simulink model "ps_isop_rail"  (R2026a)
settings: Solver=ode23tb  StopTime=param.sim.simlength  FixedStep=param.glb_time.tc  MaxStep=param.glb_time.tc
values from neighbouring files (symbols this model uses):
  param = struct()    [init_model.m]
libraries: fl_lib x49, nesl_utility x38, full_bridge_ideal_switch x4, single_phase_transformer x4, pi_ctrl x3, full_bridge_diode_rectifier x2, lithium_ion_battery x1, full_bridge_zvs_pwm_modulator x1, discrete_time_low_pass_filter x1
(part 1 of 2)
settings Model: SimulationMode=accelerator  Creator=dbagn  LastModifiedBy=dbagn
settings SolverCC: NumberNewtonIterations=3.0  ZeroCrossControl=DisableAll  SolverResetMethod=Robust
settings SFSimCC: CustomCodeUndefinedFunction=ThrowError  DefaultCustomCodeDeterministicFunctions=All
settings SFSimCC: SimCustomHeaderCode=|
  | #include "rpi.h"
  | #include "mavgflt.h"
  | #include "mavgflt_simulink.h"
  | #include "mavgflts.h"
  | #include "mavgflts_simulink.h"
  | #include "dsmavgflt.h"
  | #include "dsmavgflt_simulink.h"
  | #include "bemf_obsv.h"
  | #include "bemf_obsv_simulink.h"
  | #include "bemf_obsv_load_est.h"
  | #include "bemf_obsv_load_est_simulink.h"
  | #include "dqvector_pi.h"
  | #include "dqvector_pi_simulink.h"
  | #include "sv_pwm_simulink.h"
  | #include "sv_pwm.h"
  | #include "sv_pwm_cm_simulink.h"
  | #include "sv_pwm_cm.h"
  | #include "first_harmonic_tracker.h"
  | #include "first_harmonic_tracker_simulink.h"
  | #include "dqpll_thyr.h"
  | #include "dqpll_thyr_simulink.h"
  | #include "dqpll_grid.h"
  | #include "dqpll_grid_simulink.h"
  | #include "linear_double_integrator_observer_simulink.h"
  | #include "linear_double_integrator_observer.h"
settings SFSimCC: SimUserSources=|
  | "rpi.c"
  | "mavgflt_simulink.c"
  | "mavgflt.c"
  | "mavgflts_simulink.c"
  | "mavgflts.c"
  | "dsmavgflt_simulink.c"
  | "dsmavgflt.c"
  | "bemf_obsv_simulink.c"
  | "bemf_obsv.c"
  | "bemf_obsv_load_est_simulink.c"
  | "bemf_obsv_load_est.c"
  | "dqvector_pi.c"
  | "dqvector_pi_simulink.c"
  | "sv_pwm_simulink.c"
  | "sv_pwm.c"
  | "sv_pwm_cm_simulink.c"
  | "sv_pwm_cm.c"
  | "first_harmonic_tracker_simulink.c"
  | "first_harmonic_tracker.c"
  | "dqpll_thyr_simulink.c"
  | "dqpll_thyr.c"
  | "dqpll_grid_simulink.c"
  | "dqpll_grid.c"
  | "linear_double_integrator_observer_simulink.c"
  | "linear_double_integrator_observer.c"
settings SFSimCC: SimUserIncludeDirs=|
  | include
  | src
settings SimscapeCC: SimscapeNominalValues="[{\"value\":\"1\",\"unit\":\"A\"},{\"value\":\"1\",\"unit\":\"bar\"},{\"value\":\"1\",\"unit\":\"cm^2\"},{\"value\":\"1\",\"unit\":\"cm^3/s\"},{\"value\":\"1\",\"unit\":\"kJ/kg\"},{\"value\":\"1\",\"unit\":\"kW\"},{\"value\":\"1\",\"unit\":\"l\"},{\"value\":\"1\",\"unit\":\"N\"},{\"value\":\"1\",\"unit\":\"N*m\"},{\"value\":\"1\",\"unit\":\"V\"}]"  SimscapeLogType=none  SimscapeLogDataHistory=5000.0

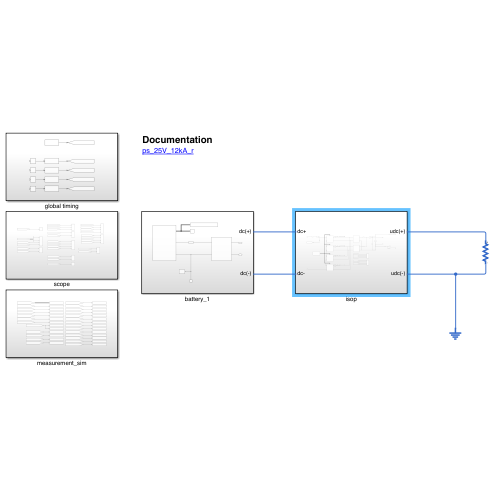
[thumbnail: Simulink's stored preview of the top-level diagram]
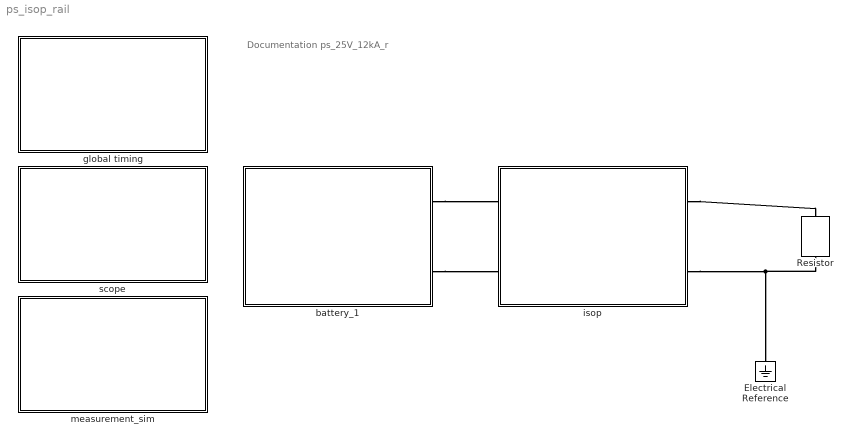
== system ps_isop_rail ==
  note: Documentation
      | ps_25V_12kA_r
  Electrical Reference : fl_lib/Electrical/Electrical Elements/Electrical Reference
  Resistor : fl_lib/Electrical/Electrical Elements/Resistor  R=param.load.rload Ohm  i_specify=off  i_priority=None  i=0 A  i_nominal_specify=off  i_nominal_value=1  i_nominal_unit=A  v_specify=off  v_priority=None  v=0 V  v_nominal_specify=off  v_nominal_value=1  v_nominal_unit=V
  battery_1 : Subsystem
  global timing : Subsystem
  isop : Subsystem
  measurement_sim : Subsystem
  scope : Subsystem
  connections:
  Resistor/RConn1 -- isop/RConn2 -- Electrical Reference/LConn1
  battery_1/RConn1 -- isop/LConn1
  battery_1/RConn2 -- isop/LConn2
  isop/RConn1 -- Resistor/LConn1

== system ps_isop_rail/battery_1 ==
  Electrical Reference : fl_lib/Electrical/Electrical Elements/Electrical Reference
  Inductor : fl_lib/Electrical/Electrical Elements/Inductor  l=param.battery.L_line H  r=0 Ohm  g=1e-9 1/Ohm  i_specify=off  i_priority=None  i=0 A  i_nominal_specify=off  i_nominal_value=1  i_nominal_unit=A  v_specify=off  v_priority=None  v=0 V  v_nominal_specify=off  v_nominal_value=1  v_nominal_unit=V  i_L_specify=off  i_L_priority=High  i_L=0 A  i_L_nominal_specify=off  i_L_nominal_value=1  i_L_nominal_unit=A
  Solver Configuration : nesl_utility/Solver Configuration  PhysicalDomain=network_engine_domain  SubClassName=solver  LeftPortType=input  RightPortType=generic  Tones=[]  Harmonics=[]  SimulateNoise=off  Profile=off  UseLocalSampling=off  EnableSwitchedLinearOptims=on  FrequencyDomain=off  UseCCode=off  RelTol=0.001  AbsTol=0.001  MinStep=1e-09  ToWorkspace=off  RevertToSquareIcSolve=off  NumHomotopyIterations=100  PhasorMode=off  PhasorModeNumHarmonics=1  ConsistencySolver=NEWTON_FTOL  CanonicalOrdering=UNORDERED  OptimizeIntermediates=UNOPTIMIZED  IndexReductionMethod=DerivativeReplacement  DoDC=on  ResidualTolerance=1e-3  ConsistencyTolSource=GLOBAL  ConsistencyAbsTol=0.001  ConsistencyRelTol=0.001  ConsistencyTolFactor=0.001  UseLocalSolver=on  LocalSolverChoice=NE_BACKWARD_EULER_ADVANCER  ResolveIndetEquations=on  FunctionEvalNumThread=1  LocalSolverSampleTime=param.glb_time.tc  DoFixedCost=on  MaxNonlinIter=param.sim.nonlinear_iterations  MaxModeIter=2  ComputeImpulses=off  ImpulseIterations=2  LinearAlgebra=auto  LinearAlgebraNumThread=0  EquationFormulation=NE_TIME_EF  DelaysMemoryBudget=1024  AutomaticFiltering=on  FilteringTimeConstant=0.001  PartitionStorageMethod=AS_NEEDED  PartitionMemoryBudget=1024  PartitionMethod=ROBUST  MultibodyUseLocalSolver=off  MultibodyLocalSolverChoice=ODE1  MultibodyLocalSolverSampleTime=0.001
  To Workspace14 : ToWorkspace  VariableName=battery_1_data_sim  SampleTime=param.glb_time.tc
      settings: MaxDataPoints=param.glb_time.Nc  Decimation=param.glb_time.decimation_tc
  lithium ion battery : Scope
      settings: ActiveDisplayYMinimum=-808.27997881012811  ActiveDisplayYMaximum=1287.7546757937268  DataLoggingVariableName=ScopeData3
  lithium_ion_battery : lithium_ion_battery/lithium_ion_battery  Q=param.battery.pack_1.Q  number_of_cells=param.battery.pack_1.number_of_cells  E_1=param.battery.pack_1.E_1  E0=param.battery.pack_1.E0  E1=param.battery.pack_1.E1  E2=param.battery.pack_1.E2  E3=param.battery.pack_1.E3  Elog=param.battery.pack_1.Elog  R0=param.battery.pack_1.R0  R1=param.battery.pack_1.R1  C1=param.battery.pack_1.C1  M=param.battery.pack_1.M  alpha=param.battery.pack_1.alpha  soc_init=param.battery.pack_1.soc_init  ts_battery=param.glb_time.ts_dab  q1Kalman=param.battery.pack_1.q1Kalman  q2Kalman=param.battery.pack_1.q2Kalman  q3Kalman=param.battery.pack_1.q3Kalman  rKalman=param.battery.pack_1.rKalman  tc=param.glb_time.tc  enable_white_noise_m=0
  single_phase_ui_measure : Subsystem
  dc(+) : PMIOPort  Side=Right
  dc(-) : PMIOPort  Port=2  Side=Right
  wires:
  lithium_ion_battery/1 -> To Workspace14/1, lithium ion battery/1
  connections:
  Solver Configuration/RConn1 -- lithium_ion_battery/RConn2 -- single_phase_ui_measure/LConn2 -- Electrical Reference/LConn1
  single_phase_ui_measure/RConn1 -- dc(+)/RConn1
  Inductor/LConn1 -- lithium_ion_battery/RConn1
  dc(-)/RConn1 -- single_phase_ui_measure/RConn2
  single_phase_ui_measure/LConn1 -- Inductor/RConn1

== system ps_isop_rail/global timing ==
  Unit Delay{1..4} (4 alike) : UnitDelay  SampleTime=param.glb_time.tc
  time_fbc1 : Subsystem  mask{k=1}
      mask prompts: k "Time Gain"
      mask Display:
      | disp('time-gen');
      | port_label('input', 1, 'crt');
      | port_label('output', 1, 'tout');
  time_fbc2 : Subsystem  mask{k=1}
      mask prompts: k "Time Gain"
      mask Display:
      | disp('time-gen');
      | port_label('input', 1, 'crt');
      | port_label('output', 1, 'tout');
  time_fbc3 : Subsystem  mask{k=1}
      mask prompts: k "Time Gain"
      mask Display:
      | disp('time-gen');
      | port_label('input', 1, 'crt');
      | port_label('output', 1, 'tout');
  time_fbc4 : Subsystem  mask{k=1}
      mask prompts: k "Time Gain"
      mask Display:
      | disp('time-gen');
      | port_label('input', 1, 'crt');
      | port_label('output', 1, 'tout');
  time_master : Subsystem  mask{k=1}
      mask prompts: k "Time Gain"
      mask Display:
      | disp('time-gen');
      | port_label('output', 1, 'tout');
  tag scope: time_isop_rail_module_1=global, time_isop_rail_module_2=global, time_isop_rail_module_3=global, time_isop_rail_module_4=global, time_master=global
  wires:
  time_master/1(Out1) -> [time_master]
  Unit Delay4/1 -> time_fbc1/1(correction_time)
  time_fbc1/1(Out1) -> [time_isop_rail_module_1]
  time_fbc2/1(Out1) -> [time_isop_rail_module_2]
  Unit Delay1/1 -> time_fbc2/1(correction_time)
  Unit Delay2/1 -> time_fbc3/1(correction_time)
  time_fbc3/1(Out1) -> [time_isop_rail_module_3]
  time_fbc4/1(Out1) -> [time_isop_rail_module_4]
  Unit Delay3/1 -> time_fbc4/1(correction_time)

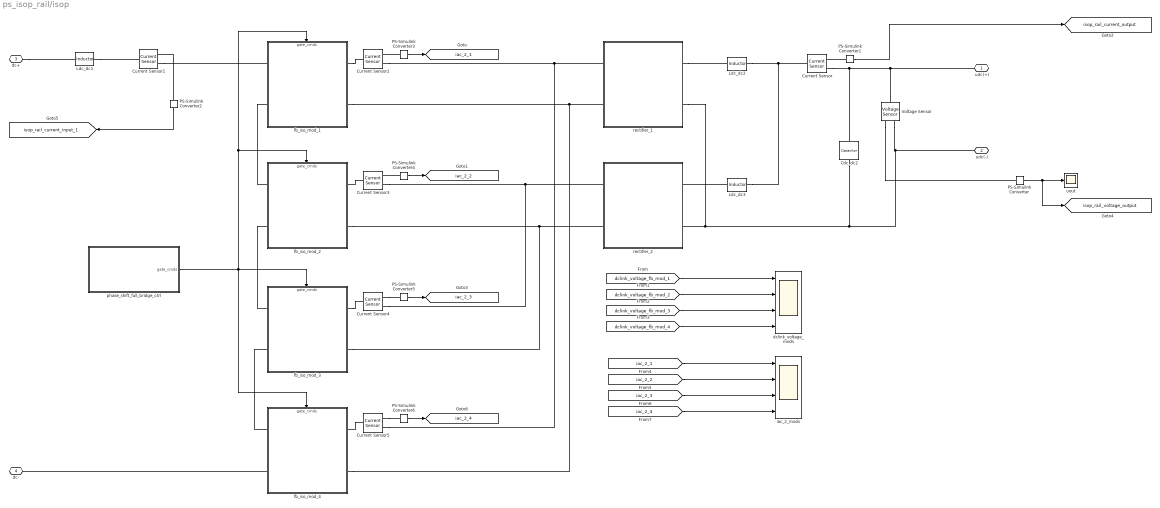
== system ps_isop_rail/isop ==
  Cdc_dc2 : fl_lib/Electrical/Electrical Elements/Capacitor  c=param.isop_rail.hw.Cdc_dc2 F  r=param.isop_rail.hw.RCdc_dc2 Ohm  g=0 1/Ohm  i_specify=off  i_priority=None  i=0 A  i_nominal_specify=off  i_nominal_value=1  i_nominal_unit=A  v_specify=off  v_priority=None  v=0 V  v_nominal_specify=off  v_nominal_value=1  v_nominal_unit=V  vc_specify=off  vc_priority=High  vc=0 V  vc_nominal_specify=off  vc_nominal_value=1  vc_nominal_unit=V
  Current Sensor{,1..5} (6 alike) : fl_lib/Electrical/Electrical Sensors/Current Sensor
  Ldc_dc1 : fl_lib/Electrical/Electrical Elements/Inductor  l=param.isop_rail.hw.Ldc_dc1 H  r=param.isop_rail.hw.RLdc_dc1 Ohm  g=1e-9 1/Ohm  i_specify=off  i_priority=None  i=0 A  i_nominal_specify=off  i_nominal_value=1  i_nominal_unit=A  v_specify=off  v_priority=None  v=0 V  v_nominal_specify=off  v_nominal_value=1  v_nominal_unit=V  i_L_specify=off  i_L_priority=High  i_L=0 A  i_L_nominal_specify=off  i_L_nominal_value=1  i_L_nominal_unit=A
  Ldc_dc2 : fl_lib/Electrical/Electrical Elements/Inductor  l=param.isop_rail.hw.Ldc_dc2 H  r=param.isop_rail.hw.RLdc_dc2 Ohm  g=1e-9 1/Ohm  i_specify=off  i_priority=None  i=0 A  i_nominal_specify=off  i_nominal_value=1  i_nominal_unit=A  v_specify=off  v_priority=None  v=0 V  v_nominal_specify=off  v_nominal_value=1  v_nominal_unit=V  i_L_specify=off  i_L_priority=High  i_L=0 A  i_L_nominal_specify=off  i_L_nominal_value=1  i_L_nominal_unit=A
  Ldc_dc3 : fl_lib/Electrical/Electrical Elements/Inductor  l=param.isop_rail.hw.Ldc_dc2 H  r=param.isop_rail.hw.RLdc_dc2 Ohm  g=1e-9 1/Ohm  i_specify=off  i_priority=None  i=0 A  i_nominal_specify=off  i_nominal_value=1  i_nominal_unit=A  v_specify=off  v_priority=None  v=0 V  v_nominal_specify=off  v_nominal_value=1  v_nominal_unit=V  i_L_specify=off  i_L_priority=High  i_L=0 A  i_L_nominal_specify=off  i_L_nominal_value=1  i_L_nominal_unit=A
  PS-Simulink Converter : nesl_utility/PS-Simulink Converter  PhysicalDomain=network_engine_domain  SubClassName=ps_output  LeftPortType=input  RightPortType=output  PseudoPeriodic=off  Frequencies=[]  VectorFormat=1-D array  Unit=V  AffineConversion=off
  PS-Simulink Converter{1..6} (6 alike) : nesl_utility/PS-Simulink Converter  PhysicalDomain=network_engine_domain  SubClassName=ps_output  LeftPortType=input  RightPortType=output  PseudoPeriodic=off  Frequencies=[]  VectorFormat=1-D array  Unit=A  AffineConversion=off
  Voltage Sensor : fl_lib/Electrical/Electrical Sensors/Voltage Sensor
  dclink_voltage_mods : Scope  NumInputPorts=4
      settings: ActiveDisplayYMinimum=1145.0339874920662  ActiveDisplayYMaximum=1193.3115786919072  DataLoggingVariableName=ScopeData4
  fb_iso_mod_1 : Subsystem
      settings: PortSchema="{\"entries\":[{\"content\":{\"sides\":[{\"content\":{\"connectorIds\":[\"In1\"]},\"type\":\"ConnectorPlacement.EquallySpacedRectSide\",\"uuid\":\"64125d2e-071e-4a4e-b242-e657f601aa6a\"},{\"content\":{\"side\":\"RIGHT\"},\"type\":\"ConnectorPlacement.EquallySpacedRectSide\",\"uuid\":\"9a259ce9-24e1-42ff-bc7d-5330e45b8a59\"},{\"content\":{\"connectorIds\":[\"LConn1\",\"LConn2\"],\"side\":\"TOP\"},\"type\":\"ConnectorPlacement.EquallySpacedRectSide\",\"uuid\":\"1c5aed3d-154a-406e-b3ed-8c68c35c38eb\"},{\"content\":{\"connectorIds\":[\"RConn1\",\"RConn2\"],\"side\":\"BOTTOM\"},\"type\":\"ConnectorPlacement.EquallySpacedRectSide\",\"uuid\":\"13746cdd-68e5-420a-ac86-8b06f3878da4\"}]},\"type\":\"ConnectorPlacement.EquallySpacedConnector\",\"uuid\":\"313792d0-2c30-49a3-9612-dddd30dbc396\"}],\"packageUris\":[\"http://schema.mathworks.com/mf0/Connector/R2020b\"],\"version\":\"1.0\"}"
  fb_iso_mod_2 : Subsystem
      settings: PortSchema="{\"entries\":[{\"content\":{\"sides\":[{\"content\":{\"connectorIds\":[\"In1\"]},\"type\":\"ConnectorPlacement.EquallySpacedRectSide\",\"uuid\":\"64125d2e-071e-4a4e-b242-e657f601aa6a\"},{\"content\":{\"side\":\"RIGHT\"},\"type\":\"ConnectorPlacement.EquallySpacedRectSide\",\"uuid\":\"9a259ce9-24e1-42ff-bc7d-5330e45b8a59\"},{\"content\":{\"connectorIds\":[\"LConn1\",\"LConn2\"],\"side\":\"TOP\"},\"type\":\"ConnectorPlacement.EquallySpacedRectSide\",\"uuid\":\"1c5aed3d-154a-406e-b3ed-8c68c35c38eb\"},{\"content\":{\"connectorIds\":[\"RConn1\",\"RConn2\"],\"side\":\"BOTTOM\"},\"type\":\"ConnectorPlacement.EquallySpacedRectSide\",\"uuid\":\"13746cdd-68e5-420a-ac86-8b06f3878da4\"}]},\"type\":\"ConnectorPlacement.EquallySpacedConnector\",\"uuid\":\"313792d0-2c30-49a3-9612-dddd30dbc396\"}],\"packageUris\":[\"http://schema.mathworks.com/mf0/Connector/R2020b\"],\"version\":\"1.0\"}"
  fb_iso_mod_3 : Subsystem
      settings: PortSchema="{\"entries\":[{\"content\":{\"sides\":[{\"content\":{\"connectorIds\":[\"In1\"]},\"type\":\"ConnectorPlacement.EquallySpacedRectSide\",\"uuid\":\"64125d2e-071e-4a4e-b242-e657f601aa6a\"},{\"content\":{\"side\":\"RIGHT\"},\"type\":\"ConnectorPlacement.EquallySpacedRectSide\",\"uuid\":\"9a259ce9-24e1-42ff-bc7d-5330e45b8a59\"},{\"content\":{\"connectorIds\":[\"LConn1\",\"LConn2\"],\"side\":\"TOP\"},\"type\":\"ConnectorPlacement.EquallySpacedRectSide\",\"uuid\":\"1c5aed3d-154a-406e-b3ed-8c68c35c38eb\"},{\"content\":{\"connectorIds\":[\"RConn1\",\"RConn2\"],\"side\":\"BOTTOM\"},\"type\":\"ConnectorPlacement.EquallySpacedRectSide\",\"uuid\":\"13746cdd-68e5-420a-ac86-8b06f3878da4\"}]},\"type\":\"ConnectorPlacement.EquallySpacedConnector\",\"uuid\":\"313792d0-2c30-49a3-9612-dddd30dbc396\"}],\"packageUris\":[\"http://schema.mathworks.com/mf0/Connector/R2020b\"],\"version\":\"1.0\"}"
  fb_iso_mod_4 : Subsystem
      settings: PortSchema="{\"entries\":[{\"content\":{\"sides\":[{\"content\":{\"connectorIds\":[\"In1\"]},\"type\":\"ConnectorPlacement.EquallySpacedRectSide\",\"uuid\":\"64125d2e-071e-4a4e-b242-e657f601aa6a\"},{\"content\":{\"side\":\"RIGHT\"},\"type\":\"ConnectorPlacement.EquallySpacedRectSide\",\"uuid\":\"9a259ce9-24e1-42ff-bc7d-5330e45b8a59\"},{\"content\":{\"connectorIds\":[\"LConn1\",\"LConn2\"],\"side\":\"TOP\"},\"type\":\"ConnectorPlacement.EquallySpacedRectSide\",\"uuid\":\"1c5aed3d-154a-406e-b3ed-8c68c35c38eb\"},{\"content\":{\"connectorIds\":[\"RConn1\",\"RConn2\"],\"side\":\"BOTTOM\"},\"type\":\"ConnectorPlacement.EquallySpacedRectSide\",\"uuid\":\"13746cdd-68e5-420a-ac86-8b06f3878da4\"}]},\"type\":\"ConnectorPlacement.EquallySpacedConnector\",\"uuid\":\"313792d0-2c30-49a3-9612-dddd30dbc396\"}],\"packageUris\":[\"http://schema.mathworks.com/mf0/Connector/R2020b\"],\"version\":\"1.0\"}"
  iac_2_mods : Scope  NumInputPorts=4
      settings: ActiveDisplayYMinimum=-468.571106856033  ActiveDisplayYMaximum=468.19314645491767  DataLoggingVariableName=ScopeData5
  phase_shift_full_bridge_ctrl : Subsystem
  rectifier_1 : Subsystem
  rectifier_2 : Subsystem
  uout : Scope
      settings: ActiveDisplayYMinimum=-94.552187389541785  ActiveDisplayYMaximum=850.96968650587621
  udc(+) : PMIOPort  Side=Right
  udc(-) : PMIOPort  Port=2  Side=Right
  dc+ : PMIOPort  Port=3  Side=Left
  dc- : PMIOPort  Port=4  Side=Left
  tag scope: iac_2_1=global, iac_2_2=global, iac_2_3=global, iac_2_4=global, isop_rail_current_input_1=global, isop_rail_current_output=global, isop_rail_voltage_output=global
  wires:
  phase_shift_full_bridge_ctrl/1(gate_cmds) -> fb_iso_mod_4/1(gate_cmds), fb_iso_mod_3/1(gate_cmds), fb_iso_mod_2/1(gate_cmds), fb_iso_mod_1/1(gate_cmds)
  PS-Simulink Converter/1 -> [isop_rail_voltage_output], uout/1
  [dclink_voltage_fb_mod_4] -> dclink_voltage_mods/4
  [dclink_voltage_fb_mod_3] -> dclink_voltage_mods/3
  [dclink_voltage_fb_mod_2] -> dclink_voltage_mods/2
  [dclink_voltage_fb_mod_1] -> dclink_voltage_mods/1
  PS-Simulink Converter1/1 -> [isop_rail_current_output]
  PS-Simulink Converter2/1 -> [isop_rail_current_input_1]
  PS-Simulink Converter3/1 -> [iac_2_1]
  PS-Simulink Converter4/1 -> [iac_2_2]
  PS-Simulink Converter5/1 -> [iac_2_3]
  PS-Simulink Converter6/1 -> [iac_2_4]
  [iac_2_4] -> iac_2_mods/4
  [iac_2_3] -> iac_2_mods/3
  [iac_2_2] -> iac_2_mods/2
  [iac_2_1] -> iac_2_mods/1
  connections:
  fb_iso_mod_2/LConn1 -- fb_iso_mod_1/LConn2
  fb_iso_mod_3/LConn1 -- fb_iso_mod_2/LConn2
  fb_iso_mod_4/LConn1 -- fb_iso_mod_3/LConn2
  fb_iso_mod_4/LConn2 -- dc-/RConn1
  Current Sensor3/RConn2 -- Current Sensor4/RConn2 -- rectifier_2/LConn1
  rectifier_2/LConn2 -- fb_iso_mod_3/RConn2 -- fb_iso_mod_2/RConn2
  Current Sensor2/RConn2 -- Current Sensor5/RConn2 -- rectifier_1/LConn1
  fb_iso_mod_1/RConn2 -- fb_iso_mod_4/RConn2 -- rectifier_1/LConn2
  udc(+)/RConn1 -- Current Sensor/RConn2 -- Cdc_dc2/LConn1 -- Voltage Sensor/LConn1
  dc+/RConn1 -- Ldc_dc1/LConn1
  Voltage Sensor/RConn1 -- PS-Simulink Converter/LConn1
  Ldc_dc2/RConn1 -- Ldc_dc3/RConn1 -- Current Sensor/LConn1
  PS-Simulink Converter1/LConn1 -- Current Sensor/RConn1
  Current Sensor1/RConn2 -- fb_iso_mod_1/LConn1
  Ldc_dc1/RConn1 -- Current Sensor1/LConn1
  PS-Simulink Converter2/LConn1 -- Current Sensor1/RConn1
  rectifier_1/RConn1 -- Ldc_dc2/LConn1
  Voltage Sensor/RConn2 -- rectifier_1/RConn2 -- rectifier_2/RConn2 -- Cdc_dc2/RConn1 -- udc(-)/RConn1
  Ldc_dc3/LConn1 -- rectifier_2/RConn1
  fb_iso_mod_1/RConn1 -- Current Sensor2/LConn1
  Current Sensor3/LConn1 -- fb_iso_mod_2/RConn1
  fb_iso_mod_3/RConn1 -- Current Sensor4/LConn1
  Current Sensor5/LConn1 -- fb_iso_mod_4/RConn1
  PS-Simulink Converter3/LConn1 -- Current Sensor2/RConn1
  PS-Simulink Converter4/LConn1 -- Current Sensor3/RConn1
  Current Sensor4/RConn1 -- PS-Simulink Converter5/LConn1
  Current Sensor5/RConn1 -- PS-Simulink Converter6/LConn1

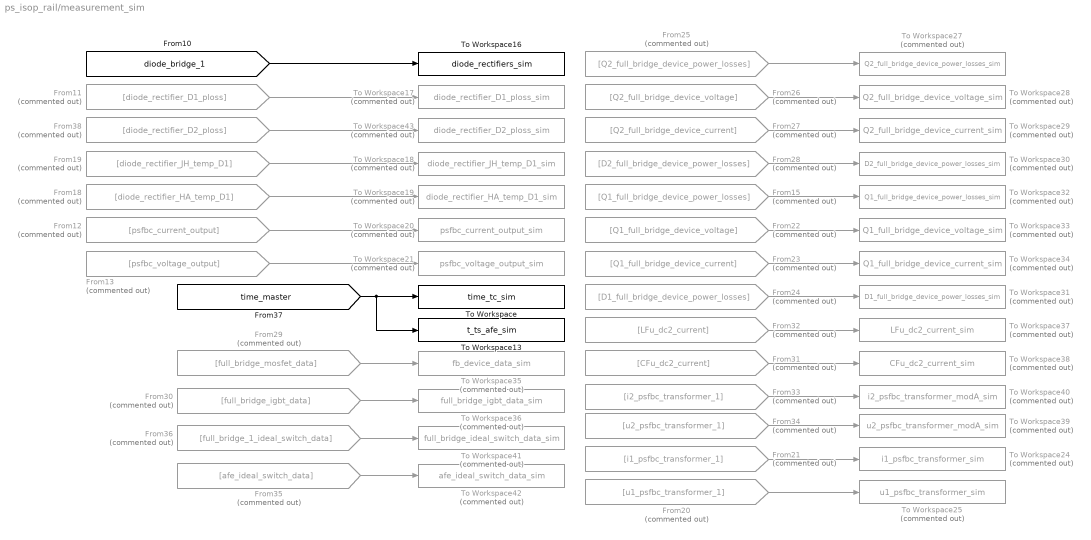
== system ps_isop_rail/measurement_sim ==
  From11 : From  Commented=on  GotoTag=diode_rectifier_D1_ploss
  From12 : From  Commented=on  GotoTag=psfbc_current_output
  From13 : From  Commented=on  GotoTag=psfbc_voltage_output
  From15 : From  Commented=on  GotoTag=Q1_full_bridge_device_power_losses
  From18 : From  Commented=on  GotoTag=diode_rectifier_HA_temp_D1
  From19 : From  Commented=on  GotoTag=diode_rectifier_JH_temp_D1
  From20 : From  Commented=on  GotoTag=u1_psfbc_transformer_1
  From21 : From  Commented=on  GotoTag=i1_psfbc_transformer_1
  From22 : From  Commented=on  GotoTag=Q1_full_bridge_device_voltage
  From23 : From  Commented=on  GotoTag=Q1_full_bridge_device_current
  From24 : From  Commented=on  GotoTag=D1_full_bridge_device_power_losses
  From25 : From  Commented=on  GotoTag=Q2_full_bridge_device_power_losses
  From26 : From  Commented=on  GotoTag=Q2_full_bridge_device_voltage
  From27 : From  Commented=on  GotoTag=Q2_full_bridge_device_current
  From28 : From  Commented=on  GotoTag=D2_full_bridge_device_power_losses
  From29 : From  Commented=on  GotoTag=full_bridge_mosfet_data
  From30 : From  Commented=on  GotoTag=full_bridge_igbt_data
  From31 : From  Commented=on  GotoTag=CFu_dc2_current
  From32 : From  Commented=on  GotoTag=LFu_dc2_current
  From33 : From  Commented=on  GotoTag=i2_psfbc_transformer_1
  From34 : From  Commented=on  GotoTag=u2_psfbc_transformer_1
  From35 : From  Commented=on  GotoTag=afe_ideal_switch_data
  From36 : From  Commented=on  GotoTag=full_bridge_1_ideal_switch_data
  From38 : From  Commented=on  GotoTag=diode_rectifier_D2_ploss
  To Workspace : ToWorkspace  VariableName=time_tc_sim  SampleTime=param.glb_time.tc
      settings: MaxDataPoints=param.glb_time.Nc  Decimation=param.glb_time.decimation_tc
  To Workspace13 : ToWorkspace  VariableName=t_ts_afe_sim  SampleTime=param.glb_time.ts_isop_rail
      settings: MaxDataPoints=param.glb_time.Ns_isop_rail
  To Workspace16 : ToWorkspace  VariableName=diode_rectifiers_sim  SampleTime=param.glb_time.tc
      settings: MaxDataPoints=param.glb_time.Nc  Decimation=param.glb_time.decimation_tc
  To Workspace17 : ToWorkspace  Commented=on  VariableName=diode_rectifier_D1_ploss_sim  SampleTime=param.glb_time.tc
      settings: MaxDataPoints=param.glb_time.Nc  Decimation=param.glb_time.decimation_tc
  To Workspace18 : ToWorkspace  Commented=on  VariableName=diode_rectifier_JH_temp_D1_sim  SampleTime=param.glb_time.tc
      settings: MaxDataPoints=param.glb_time.Nc  Decimation=param.glb_time.decimation_tc
  To Workspace19 : ToWorkspace  Commented=on  VariableName=diode_rectifier_HA_temp_D1_sim  SampleTime=param.glb_time.tc
      settings: MaxDataPoints=param.glb_time.Nc  Decimation=param.glb_time.decimation_tc
  To Workspace20 : ToWorkspace  Commented=on  VariableName=psfbc_current_output_sim  SampleTime=param.glb_time.tc
      settings: MaxDataPoints=param.glb_time.Nc  Decimation=param.glb_time.decimation_tc
  To Workspace21 : ToWorkspace  Commented=on  VariableName=psfbc_voltage_output_sim  SampleTime=param.glb_time.tc
      settings: MaxDataPoints=param.glb_time.Nc  Decimation=param.glb_time.decimation_tc
  To Workspace24 : ToWorkspace  Commented=on  VariableName=i1_psfbc_transformer_sim  SampleTime=param.glb_time.tc
      settings: MaxDataPoints=param.glb_time.Nc  Decimation=param.glb_time.decimation_tc
  To Workspace25 : ToWorkspace  Commented=on  VariableName=u1_psfbc_transformer_sim  SampleTime=param.glb_time.tc
      settings: MaxDataPoints=param.glb_time.Nc  Decimation=param.glb_time.decimation_tc
  To Workspace27 : ToWorkspace  Commented=on  VariableName=Q2_full_bridge_device_power_losses_sim  SampleTime=param.glb_time.tc
      settings: MaxDataPoints=param.glb_time.Nc  Decimation=param.glb_time.decimation_tc
  To Workspace28 : ToWorkspace  Commented=on  VariableName=Q2_full_bridge_device_voltage_sim  SampleTime=param.glb_time.tc
      settings: MaxDataPoints=param.glb_time.Nc  Decimation=param.glb_time.decimation_tc
  To Workspace29 : ToWorkspace  Commented=on  VariableName=Q2_full_bridge_device_current_sim  SampleTime=param.glb_time.tc
      settings: MaxDataPoints=param.glb_time.Nc  Decimation=param.glb_time.decimation_tc
  To Workspace30 : ToWorkspace  Commented=on  VariableName=D2_full_bridge_device_power_losses_sim  SampleTime=param.glb_time.tc
      settings: MaxDataPoints=param.glb_time.Nc  Decimation=param.glb_time.decimation_tc
  To Workspace31 : ToWorkspace  Commented=on  VariableName=D1_full_bridge_device_power_losses_sim  SampleTime=param.glb_time.tc
      settings: MaxDataPoints=param.glb_time.Nc  Decimation=param.glb_time.decimation_tc
  To Workspace32 : ToWorkspace  Commented=on  VariableName=Q1_full_bridge_device_power_losses_sim  SampleTime=param.glb_time.tc
      settings: MaxDataPoints=param.glb_time.Nc  Decimation=param.glb_time.decimation_tc
  To Workspace33 : ToWorkspace  Commented=on  VariableName=Q1_full_bridge_device_voltage_sim  SampleTime=param.glb_time.tc
      settings: MaxDataPoints=param.glb_time.Nc  Decimation=param.glb_time.decimation_tc
  To Workspace34 : ToWorkspace  Commented=on  VariableName=Q1_full_bridge_device_current_sim  SampleTime=param.glb_time.tc
      settings: MaxDataPoints=param.glb_time.Nc  Decimation=param.glb_time.decimation_tc
  To Workspace35 : ToWorkspace  Commented=on  VariableName=fb_device_data_sim  SampleTime=param.glb_time.tc
      settings: MaxDataPoints=param.glb_time.Nc  Decimation=param.glb_time.decimation_tc
  To Workspace36 : ToWorkspace  Commented=on  VariableName=full_bridge_igbt_data_sim  SampleTime=param.glb_time.tc
      settings: MaxDataPoints=param.glb_time.Nc  Decimation=param.glb_time.decimation_tc
  To Workspace37 : ToWorkspace  Commented=on  VariableName=LFu_dc2_current_sim  SampleTime=param.glb_time.tc
      settings: MaxDataPoints=param.glb_time.Nc  Decimation=param.glb_time.decimation_tc
  To Workspace38 : ToWorkspace  Commented=on  VariableName=CFu_dc2_current_sim  SampleTime=param.glb_time.tc
      settings: MaxDataPoints=param.glb_time.Nc  Decimation=param.glb_time.decimation_tc
  To Workspace39 : ToWorkspace  Commented=on  VariableName=u2_psfbc_transformer_modA_sim  SampleTime=param.glb_time.tc
      settings: MaxDataPoints=param.glb_time.Nc  Decimation=param.glb_time.decimation_tc
  To Workspace40 : ToWorkspace  Commented=on  VariableName=i2_psfbc_transformer_modA_sim  SampleTime=param.glb_time.tc
      settings: MaxDataPoints=param.glb_time.Nc  Decimation=param.glb_time.decimation_tc
  To Workspace41 : ToWorkspace  Commented=on  VariableName=full_bridge_ideal_switch_data_sim  SampleTime=param.glb_time.tc
      settings: MaxDataPoints=param.glb_time.Nc  Decimation=param.glb_time.decimation_tc
  To Workspace42 : ToWorkspace  Commented=on  VariableName=afe_ideal_switch_data_sim  SampleTime=param.glb_time.tc
      settings: MaxDataPoints=param.glb_time.Nc  Decimation=param.glb_time.decimation_tc
  To Workspace43 : ToWorkspace  Commented=on  VariableName=diode_rectifier_D2_ploss_sim  SampleTime=param.glb_time.tc
      settings: MaxDataPoints=param.glb_time.Nc  Decimation=param.glb_time.decimation_tc
  wires:
  [time_master] -> To Workspace13/1, To Workspace/1
  [diode_bridge_1] -> To Workspace16/1
  From19/1 -> To Workspace18/1
  From11/1 -> To Workspace17/1
  From18/1 -> To Workspace19/1
  From12/1 -> To Workspace20/1
  From13/1 -> To Workspace21/1
  From21/1 -> To Workspace24/1
  From20/1 -> To Workspace25/1
  From25/1 -> To Workspace27/1
  From26/1 -> To Workspace28/1
  From27/1 -> To Workspace29/1
  From15/1 -> To Workspace32/1
  From22/1 -> To Workspace33/1
  From23/1 -> To Workspace34/1
  From28/1 -> To Workspace30/1
  From24/1 -> To Workspace31/1
  From29/1 -> To Workspace35/1
  From30/1 -> To Workspace36/1
  From32/1 -> To Workspace37/1
  From31/1 -> To Workspace38/1
  From34/1 -> To Workspace39/1
  From33/1 -> To Workspace40/1
  From36/1 -> To Workspace41/1
  From35/1 -> To Workspace42/1
  From38/1 -> To Workspace43/1

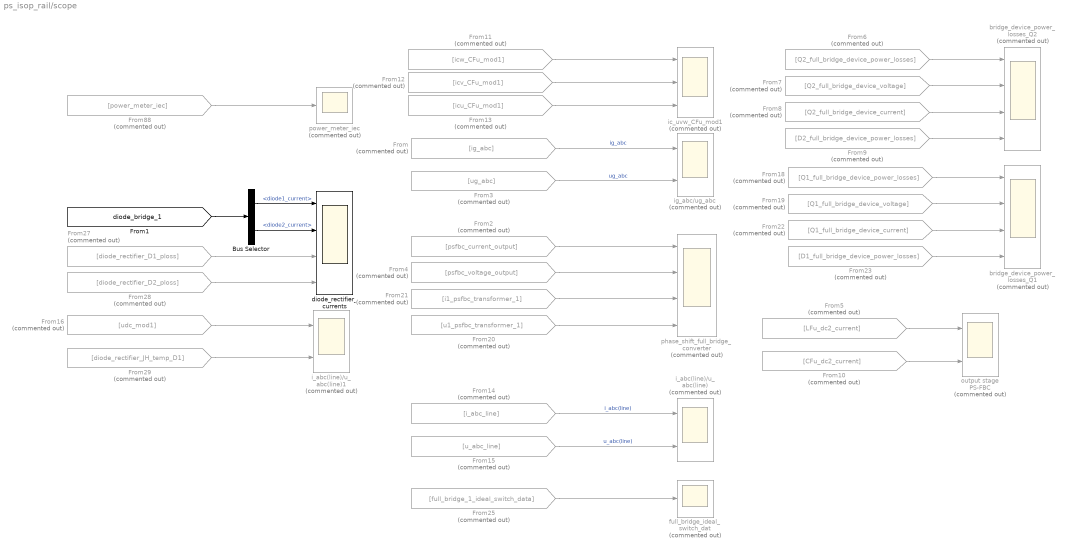
== system ps_isop_rail/scope ==
  Bus Selector : BusSelector  OutputSignals=diode1_current,diode2_current
  From : From  Commented=on  GotoTag=ig_abc
  From10 : From  Commented=on  GotoTag=CFu_dc2_current
  From11 : From  Commented=on  GotoTag=icw_CFu_mod1
  From12 : From  Commented=on  GotoTag=icv_CFu_mod1
  From13 : From  Commented=on  GotoTag=icu_CFu_mod1
  From14 : From  Commented=on  GotoTag=i_abc_line
  From15 : From  Commented=on  GotoTag=u_abc_line
  From16 : From  Commented=on  GotoTag=udc_mod1
  From18 : From  Commented=on  GotoTag=Q1_full_bridge_device_power_losses
  From19 : From  Commented=on  GotoTag=Q1_full_bridge_device_voltage
  From2 : From  Commented=on  GotoTag=psfbc_current_output
  From20 : From  Commented=on  GotoTag=u1_psfbc_transformer_1
  From21 : From  Commented=on  GotoTag=i1_psfbc_transformer_1
  From22 : From  Commented=on  GotoTag=Q1_full_bridge_device_current
  From23 : From  Commented=on  GotoTag=D1_full_bridge_device_power_losses
  From25 : From  Commented=on  GotoTag=full_bridge_1_ideal_switch_data
  From27 : From  Commented=on  GotoTag=diode_rectifier_D1_ploss
  From28 : From  Commented=on  GotoTag=diode_rectifier_D2_ploss
  From29 : From  Commented=on  GotoTag=diode_rectifier_JH_temp_D1
  From3 : From  Commented=on  GotoTag=ug_abc
  From4 : From  Commented=on  GotoTag=psfbc_voltage_output
  From5 : From  Commented=on  GotoTag=LFu_dc2_current
  From6 : From  Commented=on  GotoTag=Q2_full_bridge_device_power_losses
  From7 : From  Commented=on  GotoTag=Q2_full_bridge_device_voltage
  From8 : From  Commented=on  GotoTag=Q2_full_bridge_device_current
  From88 : From  Commented=on  GotoTag=power_meter_iec
  From9 : From  Commented=on  GotoTag=D2_full_bridge_device_power_losses
  bridge_device_power_losses_Q1 : Scope  Commented=on  NumInputPorts=4
      settings: SampleTime=param.glb_time.tc  ActiveDisplayYMinimum=-132.81353179927618  ActiveDisplayYMaximum=1178.2847224343986  DataLoggingVariableName=ScopeData23
  bridge_device_power_losses_Q2 : Scope  Commented=on  NumInputPorts=4
      settings: SampleTime=param.glb_time.tc  ActiveDisplayYMinimum=-102.91748468374873  ActiveDisplayYMaximum=909.22247743852836  DataLoggingVariableName=ScopeData20
  diode_rectifier_currents : Scope  NumInputPorts=4
      settings: ActiveDisplayString=3  ActiveDisplayYMinimum=15269.321807853252  ActiveDisplayYMaximum=15276.006477439711  DataLoggingVariableName=ScopeData11
  full_bridge_ideal_switch_dat : Scope  Commented=on
      settings: SampleTime=param.glb_time.tc  ActiveDisplayYMinimum=-185.80082711442992  ActiveDisplayYMaximum=1530.3864871069391  DataLoggingVariableName=ScopeData25
  i_abc(line)/u_abc(line) : Scope  Commented=on  NumInputPorts=2
      settings: SampleTime=param.glb_time.tc  ActiveDisplayYMinimum=-489.89794788487484  ActiveDisplayYMaximum=489.89794788490036  DataLoggingVariableName=ScopeData18
  i_abc(line)/u_abc(line)1 : Scope  Commented=on  NumInputPorts=2
      settings: SampleTime=param.glb_time.tc  ActiveDisplayYMinimum=-1  ActiveDisplayYMaximum=1  DataLoggingVariableName=ScopeData19
  ic_uvw_CFu_mod1 : Scope  Commented=on  NumInputPorts=3
      settings: SampleTime=param.glb_time.tc  ActiveDisplayYMinimum=-250.78571798939993  ActiveDisplayYMaximum=408.17461480787006  DataLoggingVariableName=ScopeData17
  ig_abc/ug_abc : Scope  Commented=on  NumInputPorts=2
      settings: SampleTime=param.glb_time.tc  ActiveDisplayYMinimum=-494.737319512461  ActiveDisplayYMaximum=494.80225542196177  DataLoggingVariableName=ScopeData15
  output stage PS-FBC : Scope  Commented=on  NumInputPorts=2
      settings: SampleTime=param.glb_time.tc  ActiveDisplayYMinimum=-658.65362756432182  ActiveDisplayYMaximum=664.76716339933853  DataLoggingVariableName=ScopeData22
  phase_shift_full_bridge_converter : Scope  Commented=on  NumInputPorts=4
      settings: SampleTime=param.glb_time.tc  ActiveDisplayYMinimum=-1597.686541193829  ActiveDisplayYMaximum=14379.178870744465  DataLoggingVariableName=ScopeData16
  power_meter_iec : Scope  Commented=on
      settings: SampleTime=param.glb_time.tc  ActiveDisplayYMinimum=-185.80082711442992  ActiveDisplayYMaximum=1530.3864871069391  DataLoggingVariableName=ScopeData27
  wires:
  From3/1 -> ig_abc/ug_abc/2  "ug_abc"
  From/1 -> ig_abc/ug_abc/1  "ig_abc"
  From11/1 -> ic_uvw_CFu_mod1/1
  From12/1 -> ic_uvw_CFu_mod1/2
  From13/1 -> ic_uvw_CFu_mod1/3
  From14/1 -> i_abc(line)/u_abc(line)/1  "i_abc(line)"
  From15/1 -> i_abc(line)/u_abc(line)/2  "u_abc(line)"
  From16/1 -> i_abc(line)/u_abc(line)1/1
  [diode_bridge_1] -> Bus Selector/1
  From2/1 -> phase_shift_full_bridge_converter/1
  From4/1 -> phase_shift_full_bridge_converter/2
  From21/1 -> phase_shift_full_bridge_converter/3
  From20/1 -> phase_shift_full_bridge_converter/4
  Bus Selector/1 -> diode_rectifier_currents/1  "<diode1_current>"
  Bus Selector/2 -> diode_rectifier_currents/2  "<diode2_current>"
  From5/1 -> output stage PS-FBC/1
  From10/1 -> output stage PS-FBC/2
  From6/1 -> bridge_device_power_losses_Q2/1
  From7/1 -> bridge_device_power_losses_Q2/2
  From8/1 -> bridge_device_power_losses_Q2/3
  From9/1 -> bridge_device_power_losses_Q2/4
  From18/1 -> bridge_device_power_losses_Q1/1
  From19/1 -> bridge_device_power_losses_Q1/2
  From22/1 -> bridge_device_power_losses_Q1/3
  From23/1 -> bridge_device_power_losses_Q1/4
  From25/1 -> full_bridge_ideal_switch_dat/1
  From27/1 -> diode_rectifier_currents/3
  From28/1 -> diode_rectifier_currents/4
  From29/1 -> i_abc(line)/u_abc(line)1/2
  From88/1 -> power_meter_iec/1

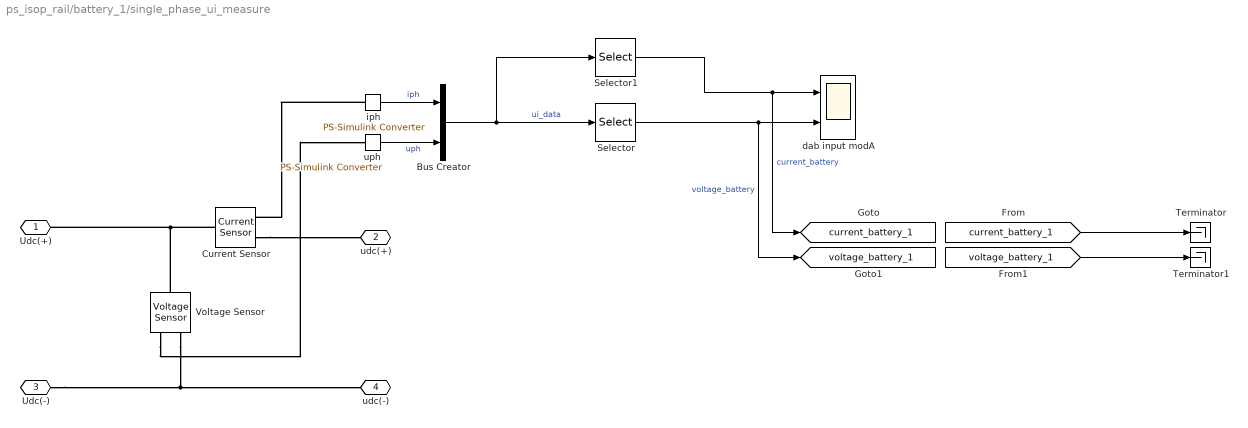
== system ps_isop_rail/battery_1/single_phase_ui_measure ==
  Bus Creator : BusCreator  Inputs=2
  Current Sensor : fl_lib/Electrical/Electrical Sensors/Current Sensor
  Selector : Selector  InputPortWidth=2  IndexOptions=Index vector (dialog)  Indices=2  OutputSizes=1
  Selector1 : Selector  InputPortWidth=2  IndexOptions=Index vector (dialog)  Indices=1  OutputSizes=1
  Terminator : Terminator
  Terminator1 : Terminator
  Voltage Sensor : fl_lib/Electrical/Electrical Sensors/Voltage Sensor
  dab input modA : Scope  NumInputPorts=2
      settings: SampleTime=param.glb_time.tc  ActiveDisplayYMinimum=4618.3089115716557  ActiveDisplayYMaximum=4703.2257607249676  DataLoggingVariableName=ScopeData2
  iph : nesl_utility/PS-Simulink Converter  PhysicalDomain=network_engine_domain  SubClassName=ps_output  LeftPortType=input  RightPortType=output  PseudoPeriodic=off  Frequencies=[]  VectorFormat=1-D array  Unit=A  AffineConversion=off
  uph : nesl_utility/PS-Simulink Converter  PhysicalDomain=network_engine_domain  SubClassName=ps_output  LeftPortType=input  RightPortType=output  PseudoPeriodic=off  Frequencies=[]  VectorFormat=1-D array  Unit=V  AffineConversion=off
  Udc(+) : PMIOPort  Side=Left
  udc(+) : PMIOPort  Port=2  Side=Right
  Udc(-) : PMIOPort  Port=3  Side=Left
  udc(-) : PMIOPort  Port=4  Side=Right
  tag scope: current_battery_1=global, voltage_battery_1=global
  wires:
  Bus Creator/1 -> Selector/1, Selector1/1  "ui_data"
  iph/1 -> Bus Creator/1  "iph"
  uph/1 -> Bus Creator/2  "uph"
  Selector1/1 -> [current_battery_1], dab input modA/1  "current_battery"
  Selector/1 -> dab input modA/2, [voltage_battery_1]  "voltage_battery"
  [current_battery_1] -> Terminator/1
  [voltage_battery_1] -> Terminator1/1
  connections:
  iph/LConn1 -- Current Sensor/RConn1
  Voltage Sensor/LConn1 -- Current Sensor/LConn1 -- Udc(+)/RConn1
  Current Sensor/RConn2 -- udc(+)/RConn1
  Voltage Sensor/RConn1 -- uph/LConn1
  Voltage Sensor/RConn2 -- Udc(-)/RConn1 -- udc(-)/RConn1

== system ps_isop_rail/global timing/time_fbc1 ==
  correction_time : Inport
  Constant : Constant
  Gain : Gain  Gain=k
  Product : Product
  Sum : Sum  Inputs=|++
  time_1 : Clock
  Out1 : Outport
  wires:
  Sum/1 -> Product/2
  Constant/1 -> Sum/2
  correction_time/1 -> Sum/1
  Product/1 -> Out1/1
  Gain/1 -> Product/1
  time_1/1 -> Gain/1

== system ps_isop_rail/global timing/time_fbc2 ==
  correction_time : Inport
  Constant : Constant
  Gain : Gain  Gain=k
  Product : Product
  Sum : Sum  Inputs=|++
  time_1 : Clock
  Out1 : Outport
  wires:
  time_1/1 -> Gain/1
  Gain/1 -> Product/1
  Product/1 -> Out1/1
  correction_time/1 -> Sum/1
  Constant/1 -> Sum/2
  Sum/1 -> Product/2

== system ps_isop_rail/global timing/time_fbc3 ==
  correction_time : Inport
  Constant : Constant
  Gain : Gain  Gain=k
  Product : Product
  Sum : Sum  Inputs=|++
  time_1 : Clock
  Out1 : Outport
  wires:
  Sum/1 -> Product/2
  Constant/1 -> Sum/2
  correction_time/1 -> Sum/1
  Product/1 -> Out1/1
  Gain/1 -> Product/1
  time_1/1 -> Gain/1

== system ps_isop_rail/global timing/time_fbc4 ==
  correction_time : Inport
  Constant : Constant
  Gain : Gain  Gain=k
  Product : Product
  Sum : Sum  Inputs=|++
  time_1 : Clock
  Out1 : Outport
  wires:
  time_1/1 -> Gain/1
  Gain/1 -> Product/1
  Product/1 -> Out1/1
  correction_time/1 -> Sum/1
  Constant/1 -> Sum/2
  Sum/1 -> Product/2

== system ps_isop_rail/global timing/time_master ==
  Gain : Gain  Gain=k
  time_1 : Clock
  Out1 : Outport
  wires:
  Gain/1 -> Out1/1
  time_1/1 -> Gain/1

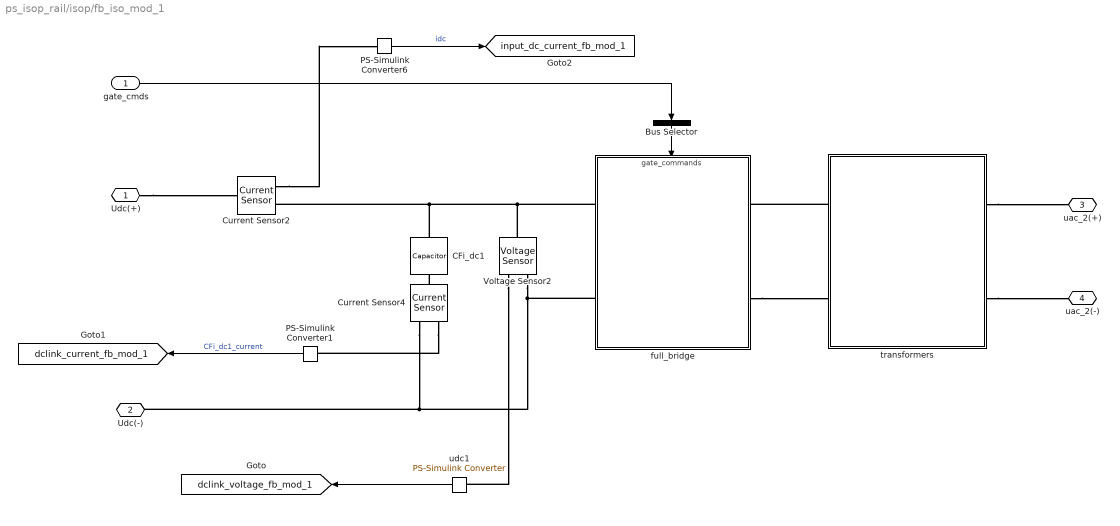
== system ps_isop_rail/isop/fb_iso_mod_1 ==
  gate_cmds : Inport
  Bus Selector : BusSelector  OutputSignals=gate_cmd_Q1,gate_cmd_Q2,gate_cmd_Q3,gate_cmd_Q4  OutputAsBus=on
  CFi_dc1 : fl_lib/Electrical/Electrical Elements/Capacitor  c=param.isop_rail.hw.Cdc_dc1 F  r=param.isop_rail.hw.RCdc_dc1 Ohm  g=0 1/Ohm  i_specify=off  i_priority=None  i=0 A  i_nominal_specify=off  i_nominal_value=1  i_nominal_unit=A  v_specify=off  v_priority=High  v=0 V  v_nominal_specify=off  v_nominal_value=1  v_nominal_unit=V  vc_specify=on  vc_priority=High  vc=0 V  vc_nominal_specify=off  vc_nominal_value=1  vc_nominal_unit=V
  Current Sensor2 : fl_lib/Electrical/Electrical Sensors/Current Sensor
  Current Sensor4 : fl_lib/Electrical/Electrical Sensors/Current Sensor
  PS-Simulink Converter1 : nesl_utility/PS-Simulink Converter  PhysicalDomain=network_engine_domain  SubClassName=ps_output  LeftPortType=input  RightPortType=output  PseudoPeriodic=off  Frequencies=[]  VectorFormat=1-D array  Unit=A  AffineConversion=on
  PS-Simulink Converter6 : nesl_utility/PS-Simulink Converter  PhysicalDomain=network_engine_domain  SubClassName=ps_output  LeftPortType=input  RightPortType=output  PseudoPeriodic=off  Frequencies=[]  VectorFormat=1-D array  Unit=A  AffineConversion=on
  Voltage Sensor2 : fl_lib/Electrical/Electrical Sensors/Voltage Sensor
  full_bridge : Subsystem
      settings: PortSchema="{\"entries\":[{\"content\":{\"sides\":[{\"content\":{\"connectorIds\":[\"LConn1\",\"LConn2\"]},\"type\":\"ConnectorPlacement.EquallySpacedRectSide\",\"uuid\":\"c872503a-61af-4937-bdf2-4de4f8645573\"},{\"content\":{\"connectorIds\":[\"RConn1\",\"RConn2\"],\"side\":\"RIGHT\"},\"type\":\"ConnectorPlacement.EquallySpacedRectSide\",\"uuid\":\"3b83f060-86a2-4569-84b5-d9f7c0485347\"},{\"content\":{\"connectorIds\":[\"In1\"],\"side\":\"TOP\"},\"type\":\"ConnectorPlacement.EquallySpacedRectSide\",\"uuid\":\"bf191d46-ce71-4d15-9dd0-24cc57253577\"}]},\"type\":\"ConnectorPlacement.EquallySpacedConnector\",\"uuid\":\"1b28ceee-25d0-45ae-a3c4-c2563f0d63ba\"}],\"packageUris\":[\"http://schema.mathworks.com/mf0/Connector/R2020b\"],\"version\":\"1.0\"}"
  transformers : Subsystem
  udc1 : nesl_utility/PS-Simulink Converter  PhysicalDomain=network_engine_domain  SubClassName=ps_output  LeftPortType=input  RightPortType=output  PseudoPeriodic=off  Frequencies=[]  VectorFormat=1-D array  Unit=V  AffineConversion=off
  Udc(+) : PMIOPort  Side=Left
  Udc(-) : PMIOPort  Port=2  Side=Left
  uac_2(+) : PMIOPort  Port=3  Side=Right
  uac_2(-) : PMIOPort  Port=4  Side=Right
  tag scope: dclink_current_fb_mod_1=global, dclink_voltage_fb_mod_1=global, input_dc_current_fb_mod_1=global
  wires:
  gate_cmds/1 -> Bus Selector/1
  PS-Simulink Converter6/1 -> [input_dc_current_fb_mod_1]  "idc"
  Bus Selector/1 -> full_bridge/1(gate_commands)
  udc1/1 -> [dclink_voltage_fb_mod_1]
  PS-Simulink Converter1/1 -> [dclink_current_fb_mod_1]  "CFi_dc1_current"
  connections:
  full_bridge/RConn2 -- Voltage Sensor2/RConn2 -- Current Sensor4/RConn2 -- Udc(-)/RConn1
  full_bridge/RConn1 -- Voltage Sensor2/LConn1 -- Current Sensor2/RConn2 -- CFi_dc1/LConn1
  Udc(+)/RConn1 -- Current Sensor2/LConn1
  Current Sensor2/RConn1 -- PS-Simulink Converter6/LConn1
  Voltage Sensor2/RConn1 -- udc1/LConn1
  Current Sensor4/LConn1 -- CFi_dc1/RConn1
  Current Sensor4/RConn1 -- PS-Simulink Converter1/LConn1
  transformers/LConn1 -- full_bridge/LConn1
  full_bridge/LConn2 -- transformers/LConn2
  transformers/RConn1 -- uac_2(+)/RConn1
  transformers/RConn2 -- uac_2(-)/RConn1

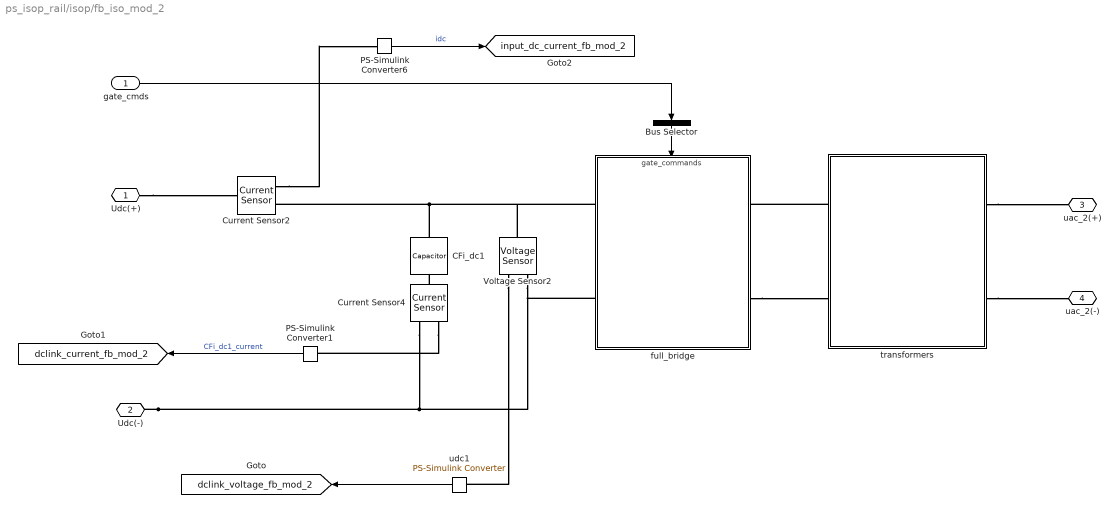
== system ps_isop_rail/isop/fb_iso_mod_2 ==
  gate_cmds : Inport
  Bus Selector : BusSelector  OutputSignals=gate_cmd_Q1,gate_cmd_Q2,gate_cmd_Q3,gate_cmd_Q4  OutputAsBus=on
  CFi_dc1 : fl_lib/Electrical/Electrical Elements/Capacitor  c=param.isop_rail.hw.Cdc_dc1 F  r=param.isop_rail.hw.RCdc_dc1 Ohm  g=0 1/Ohm  i_specify=off  i_priority=None  i=0 A  i_nominal_specify=off  i_nominal_value=1  i_nominal_unit=A  v_specify=off  v_priority=High  v=0 V  v_nominal_specify=off  v_nominal_value=1  v_nominal_unit=V  vc_specify=on  vc_priority=High  vc=0 V  vc_nominal_specify=off  vc_nominal_value=1  vc_nominal_unit=V
  Current Sensor2 : fl_lib/Electrical/Electrical Sensors/Current Sensor
  Current Sensor4 : fl_lib/Electrical/Electrical Sensors/Current Sensor
  PS-Simulink Converter1 : nesl_utility/PS-Simulink Converter  PhysicalDomain=network_engine_domain  SubClassName=ps_output  LeftPortType=input  RightPortType=output  PseudoPeriodic=off  Frequencies=[]  VectorFormat=1-D array  Unit=A  AffineConversion=on
  PS-Simulink Converter6 : nesl_utility/PS-Simulink Converter  PhysicalDomain=network_engine_domain  SubClassName=ps_output  LeftPortType=input  RightPortType=output  PseudoPeriodic=off  Frequencies=[]  VectorFormat=1-D array  Unit=A  AffineConversion=on
  Voltage Sensor2 : fl_lib/Electrical/Electrical Sensors/Voltage Sensor
  full_bridge : Subsystem
      settings: PortSchema="{\"entries\":[{\"content\":{\"sides\":[{\"content\":{\"connectorIds\":[\"LConn1\",\"LConn2\"]},\"type\":\"ConnectorPlacement.EquallySpacedRectSide\",\"uuid\":\"c872503a-61af-4937-bdf2-4de4f8645573\"},{\"content\":{\"connectorIds\":[\"RConn1\",\"RConn2\"],\"side\":\"RIGHT\"},\"type\":\"ConnectorPlacement.EquallySpacedRectSide\",\"uuid\":\"3b83f060-86a2-4569-84b5-d9f7c0485347\"},{\"content\":{\"connectorIds\":[\"In1\"],\"side\":\"TOP\"},\"type\":\"ConnectorPlacement.EquallySpacedRectSide\",\"uuid\":\"bf191d46-ce71-4d15-9dd0-24cc57253577\"}]},\"type\":\"ConnectorPlacement.EquallySpacedConnector\",\"uuid\":\"1b28ceee-25d0-45ae-a3c4-c2563f0d63ba\"}],\"packageUris\":[\"http://schema.mathworks.com/mf0/Connector/R2020b\"],\"version\":\"1.0\"}"
  transformers : Subsystem
  udc1 : nesl_utility/PS-Simulink Converter  PhysicalDomain=network_engine_domain  SubClassName=ps_output  LeftPortType=input  RightPortType=output  PseudoPeriodic=off  Frequencies=[]  VectorFormat=1-D array  Unit=V  AffineConversion=off
  Udc(+) : PMIOPort  Side=Left
  Udc(-) : PMIOPort  Port=2  Side=Left
  uac_2(+) : PMIOPort  Port=3  Side=Right
  uac_2(-) : PMIOPort  Port=4  Side=Right
  tag scope: dclink_current_fb_mod_2=global, dclink_voltage_fb_mod_2=global, input_dc_current_fb_mod_2=global
  wires:
  PS-Simulink Converter1/1 -> [dclink_current_fb_mod_2]  "CFi_dc1_current"
  udc1/1 -> [dclink_voltage_fb_mod_2]
  Bus Selector/1 -> full_bridge/1(gate_commands)
  PS-Simulink Converter6/1 -> [input_dc_current_fb_mod_2]  "idc"
  gate_cmds/1 -> Bus Selector/1
  connections:
  transformers/RConn2 -- uac_2(-)/RConn1
  transformers/RConn1 -- uac_2(+)/RConn1
  full_bridge/LConn2 -- transformers/LConn2
  transformers/LConn1 -- full_bridge/LConn1
  Current Sensor4/RConn1 -- PS-Simulink Converter1/LConn1
  Current Sensor4/LConn1 -- CFi_dc1/RConn1
  Voltage Sensor2/RConn1 -- udc1/LConn1
  Current Sensor2/RConn1 -- PS-Simulink Converter6/LConn1
  Udc(+)/RConn1 -- Current Sensor2/LConn1
  CFi_dc1/LConn1 -- Current Sensor2/RConn2 -- Voltage Sensor2/LConn1 -- full_bridge/RConn1
  Udc(-)/RConn1 -- Current Sensor4/RConn2 -- Voltage Sensor2/RConn2 -- full_bridge/RConn2

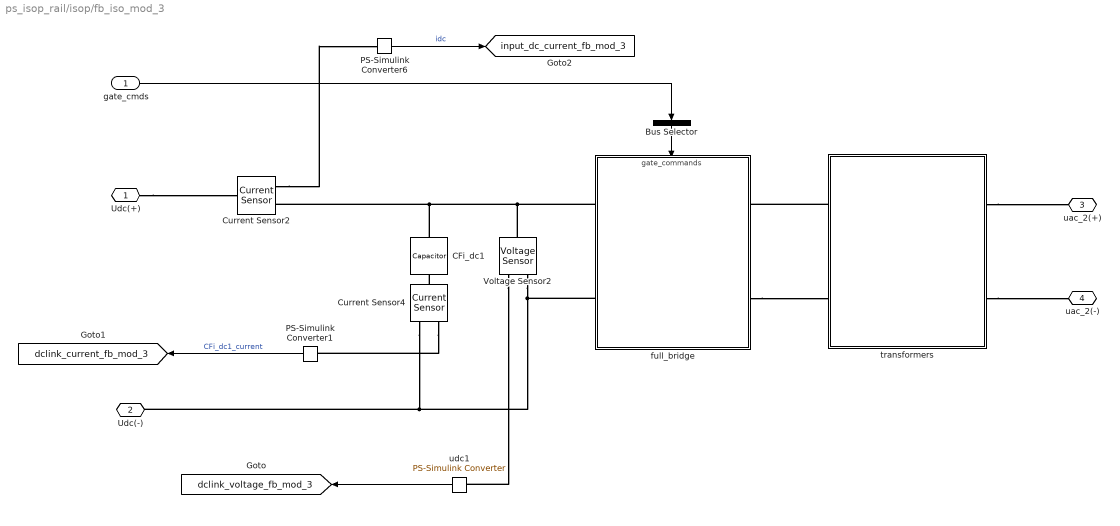
== system ps_isop_rail/isop/fb_iso_mod_3 ==
  gate_cmds : Inport
  Bus Selector : BusSelector  OutputSignals=gate_cmd_Q1,gate_cmd_Q2,gate_cmd_Q3,gate_cmd_Q4  OutputAsBus=on
  CFi_dc1 : fl_lib/Electrical/Electrical Elements/Capacitor  c=param.isop_rail.hw.Cdc_dc1 F  r=param.isop_rail.hw.RCdc_dc1 Ohm  g=0 1/Ohm  i_specify=off  i_priority=None  i=0 A  i_nominal_specify=off  i_nominal_value=1  i_nominal_unit=A  v_specify=off  v_priority=None  v=0 V  v_nominal_specify=off  v_nominal_value=1  v_nominal_unit=V  vc_specify=on  vc_priority=High  vc=0 V  vc_nominal_specify=off  vc_nominal_value=1  vc_nominal_unit=V
  Current Sensor2 : fl_lib/Electrical/Electrical Sensors/Current Sensor
  Current Sensor4 : fl_lib/Electrical/Electrical Sensors/Current Sensor
  PS-Simulink Converter1 : nesl_utility/PS-Simulink Converter  PhysicalDomain=network_engine_domain  SubClassName=ps_output  LeftPortType=input  RightPortType=output  PseudoPeriodic=off  Frequencies=[]  VectorFormat=1-D array  Unit=A  AffineConversion=on
  PS-Simulink Converter6 : nesl_utility/PS-Simulink Converter  PhysicalDomain=network_engine_domain  SubClassName=ps_output  LeftPortType=input  RightPortType=output  PseudoPeriodic=off  Frequencies=[]  VectorFormat=1-D array  Unit=A  AffineConversion=on
  Voltage Sensor2 : fl_lib/Electrical/Electrical Sensors/Voltage Sensor
  full_bridge : Subsystem
      settings: PortSchema="{\"entries\":[{\"content\":{\"sides\":[{\"content\":{\"connectorIds\":[\"LConn1\",\"LConn2\"]},\"type\":\"ConnectorPlacement.EquallySpacedRectSide\",\"uuid\":\"c872503a-61af-4937-bdf2-4de4f8645573\"},{\"content\":{\"connectorIds\":[\"RConn1\",\"RConn2\"],\"side\":\"RIGHT\"},\"type\":\"ConnectorPlacement.EquallySpacedRectSide\",\"uuid\":\"3b83f060-86a2-4569-84b5-d9f7c0485347\"},{\"content\":{\"connectorIds\":[\"In1\"],\"side\":\"TOP\"},\"type\":\"ConnectorPlacement.EquallySpacedRectSide\",\"uuid\":\"bf191d46-ce71-4d15-9dd0-24cc57253577\"}]},\"type\":\"ConnectorPlacement.EquallySpacedConnector\",\"uuid\":\"1b28ceee-25d0-45ae-a3c4-c2563f0d63ba\"}],\"packageUris\":[\"http://schema.mathworks.com/mf0/Connector/R2020b\"],\"version\":\"1.0\"}"
  transformers : Subsystem
  udc1 : nesl_utility/PS-Simulink Converter  PhysicalDomain=network_engine_domain  SubClassName=ps_output  LeftPortType=input  RightPortType=output  PseudoPeriodic=off  Frequencies=[]  VectorFormat=1-D array  Unit=V  AffineConversion=off
  Udc(+) : PMIOPort  Side=Left
  Udc(-) : PMIOPort  Port=2  Side=Left
  uac_2(+) : PMIOPort  Port=3  Side=Right
  uac_2(-) : PMIOPort  Port=4  Side=Right
  tag scope: dclink_current_fb_mod_3=global, dclink_voltage_fb_mod_3=global, input_dc_current_fb_mod_3=global
  wires:
  gate_cmds/1 -> Bus Selector/1
  PS-Simulink Converter6/1 -> [input_dc_current_fb_mod_3]  "idc"
  Bus Selector/1 -> full_bridge/1(gate_commands)
  udc1/1 -> [dclink_voltage_fb_mod_3]
  PS-Simulink Converter1/1 -> [dclink_current_fb_mod_3]  "CFi_dc1_current"
  connections:
  full_bridge/RConn2 -- Voltage Sensor2/RConn2 -- Current Sensor4/RConn2 -- Udc(-)/RConn1
  full_bridge/RConn1 -- Voltage Sensor2/LConn1 -- Current Sensor2/RConn2 -- CFi_dc1/LConn1
  Udc(+)/RConn1 -- Current Sensor2/LConn1
  Current Sensor2/RConn1 -- PS-Simulink Converter6/LConn1
  Voltage Sensor2/RConn1 -- udc1/LConn1
  Current Sensor4/LConn1 -- CFi_dc1/RConn1
  Current Sensor4/RConn1 -- PS-Simulink Converter1/LConn1
  transformers/LConn1 -- full_bridge/LConn1
  full_bridge/LConn2 -- transformers/LConn2
  transformers/RConn1 -- uac_2(+)/RConn1
  transformers/RConn2 -- uac_2(-)/RConn1

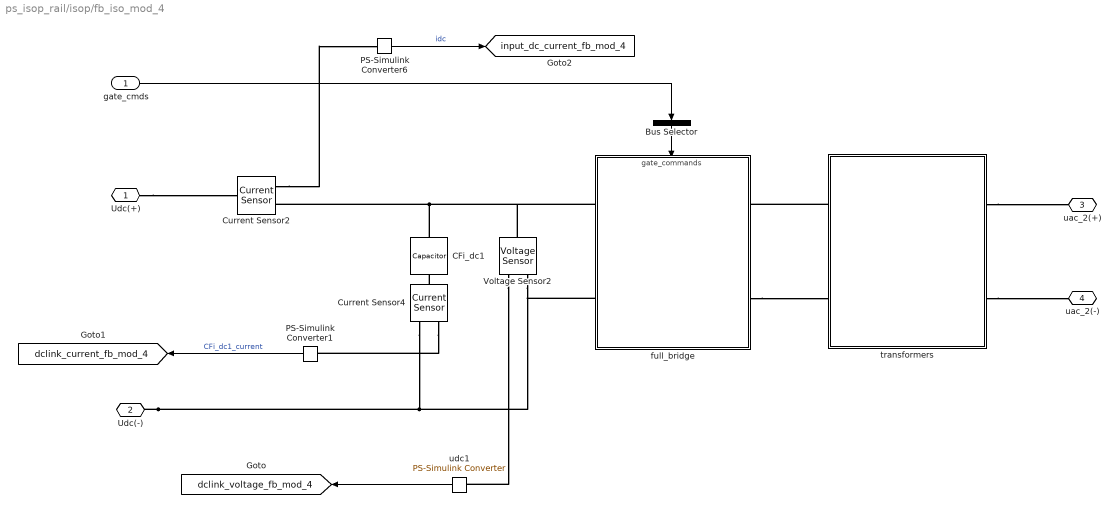
== system ps_isop_rail/isop/fb_iso_mod_4 ==
  gate_cmds : Inport
  Bus Selector : BusSelector  OutputSignals=gate_cmd_Q1,gate_cmd_Q2,gate_cmd_Q3,gate_cmd_Q4  OutputAsBus=on
  CFi_dc1 : fl_lib/Electrical/Electrical Elements/Capacitor  c=param.isop_rail.hw.Cdc_dc1 F  r=param.isop_rail.hw.RCdc_dc1 Ohm  g=0 1/Ohm  i_specify=off  i_priority=None  i=0 A  i_nominal_specify=off  i_nominal_value=1  i_nominal_unit=A  v_specify=off  v_priority=None  v=0 V  v_nominal_specify=off  v_nominal_value=1  v_nominal_unit=V  vc_specify=on  vc_priority=High  vc=0 V  vc_nominal_specify=off  vc_nominal_value=1  vc_nominal_unit=V
  Current Sensor2 : fl_lib/Electrical/Electrical Sensors/Current Sensor
  Current Sensor4 : fl_lib/Electrical/Electrical Sensors/Current Sensor
  PS-Simulink Converter1 : nesl_utility/PS-Simulink Converter  PhysicalDomain=network_engine_domain  SubClassName=ps_output  LeftPortType=input  RightPortType=output  PseudoPeriodic=off  Frequencies=[]  VectorFormat=1-D array  Unit=A  AffineConversion=on
  PS-Simulink Converter6 : nesl_utility/PS-Simulink Converter  PhysicalDomain=network_engine_domain  SubClassName=ps_output  LeftPortType=input  RightPortType=output  PseudoPeriodic=off  Frequencies=[]  VectorFormat=1-D array  Unit=A  AffineConversion=on
  Voltage Sensor2 : fl_lib/Electrical/Electrical Sensors/Voltage Sensor
  full_bridge : Subsystem
      settings: PortSchema="{\"entries\":[{\"content\":{\"sides\":[{\"content\":{\"connectorIds\":[\"LConn1\",\"LConn2\"]},\"type\":\"ConnectorPlacement.EquallySpacedRectSide\",\"uuid\":\"c872503a-61af-4937-bdf2-4de4f8645573\"},{\"content\":{\"connectorIds\":[\"RConn1\",\"RConn2\"],\"side\":\"RIGHT\"},\"type\":\"ConnectorPlacement.EquallySpacedRectSide\",\"uuid\":\"3b83f060-86a2-4569-84b5-d9f7c0485347\"},{\"content\":{\"connectorIds\":[\"In1\"],\"side\":\"TOP\"},\"type\":\"ConnectorPlacement.EquallySpacedRectSide\",\"uuid\":\"bf191d46-ce71-4d15-9dd0-24cc57253577\"}]},\"type\":\"ConnectorPlacement.EquallySpacedConnector\",\"uuid\":\"1b28ceee-25d0-45ae-a3c4-c2563f0d63ba\"}],\"packageUris\":[\"http://schema.mathworks.com/mf0/Connector/R2020b\"],\"version\":\"1.0\"}"
  transformers : Subsystem
  udc1 : nesl_utility/PS-Simulink Converter  PhysicalDomain=network_engine_domain  SubClassName=ps_output  LeftPortType=input  RightPortType=output  PseudoPeriodic=off  Frequencies=[]  VectorFormat=1-D array  Unit=V  AffineConversion=off
  Udc(+) : PMIOPort  Side=Left
  Udc(-) : PMIOPort  Port=2  Side=Left
  uac_2(+) : PMIOPort  Port=3  Side=Right
  uac_2(-) : PMIOPort  Port=4  Side=Right
  tag scope: dclink_current_fb_mod_4=global, dclink_voltage_fb_mod_4=global, input_dc_current_fb_mod_4=global
  wires:
  PS-Simulink Converter1/1 -> [dclink_current_fb_mod_4]  "CFi_dc1_current"
  udc1/1 -> [dclink_voltage_fb_mod_4]
  Bus Selector/1 -> full_bridge/1(gate_commands)
  PS-Simulink Converter6/1 -> [input_dc_current_fb_mod_4]  "idc"
  gate_cmds/1 -> Bus Selector/1
  connections:
  transformers/RConn2 -- uac_2(-)/RConn1
  transformers/RConn1 -- uac_2(+)/RConn1
  full_bridge/LConn2 -- transformers/LConn2
  transformers/LConn1 -- full_bridge/LConn1
  Current Sensor4/RConn1 -- PS-Simulink Converter1/LConn1
  Current Sensor4/LConn1 -- CFi_dc1/RConn1
  Voltage Sensor2/RConn1 -- udc1/LConn1
  Current Sensor2/RConn1 -- PS-Simulink Converter6/LConn1
  Udc(+)/RConn1 -- Current Sensor2/LConn1
  CFi_dc1/LConn1 -- Current Sensor2/RConn2 -- Voltage Sensor2/LConn1 -- full_bridge/RConn1
  Udc(-)/RConn1 -- Current Sensor4/RConn2 -- Voltage Sensor2/RConn2 -- full_bridge/RConn2
